simulink model "FSC_SCHEME"  (R2024b)
settings: Solver=FixedStepAuto  StartTime=0.0  StopTime=inf  FixedStep=0.001  RelTol=1e-3  EnableMultiTasking=on
libraries: px4Sensorslib x2, px4Peripheralslib x1
settings Model: SimulationMode=external  ExtModeTrigDuration=10  Creator=ArriGE66  LastModifiedBy=xippa
settings SolverCC: PositivePriorityOrder=on
settings OptimizationCC: EnhancedBackFolding=on  PassReuseOutputArgsAs=Individual arguments  ZeroExternalMemoryAtStartup=off  ZeroInternalMemoryAtStartup=off  MaxStackSize=64  OptimizeBlockOrder=speed  DifferentSizesBufferReuse=on  OptimizationCustomize=off  EfficientTunableParamExpr=on
settings DebuggingCC: ParameterTunabilityLossMsg=error
settings HardwareCC: ProdBitPerPointer=32  ProdBitPerSizeT=32  ProdBitPerPtrDiffT=32  ProdLargestAtomicInteger=Long  ProdLargestAtomicFloat=Double  ProdWordSize=32  ProdLongLongMode=on  ProdHWDeviceType=ARM Compatible->ARM Cortex
settings SFSimCC: MATLABDynamicMemAlloc=off  SimTargetLang=C++
settings RTWCC: Description=Embedded Coder  SystemTargetFile=ert.tlc  HardwareBoard=PX4 Cube Orange  TemplateMakefile=ert_default_tmf  Toolchain=GNU Tools for PX4 Autopilots  TargetLang=C++  GPUComputeCapability=3.5
settings CodeAppCC: ForceParamTrailComments=on  IgnoreCustomStorageClasses=off  OperatorAnnotations=on  SimulinkDataObjDesc=on  SFDataObjDesc=on  InsertBlockDesc=on
settings ERTTargetCC: SupportVariableSizeSignals=on  ExtMode=on  ExtModeTransport=3  ExtModeStaticAlloc=on  ExtModeStaticAllocSize=1024  ExtModeMexFile=ext_xcp  ExtModeMexArgs=1 COM10 3000000  ExtModeIntrfLevel=Level2 - Open  InlinedParameterPlacement=Hierarchical  DynamicArrayContainerType=coder::array

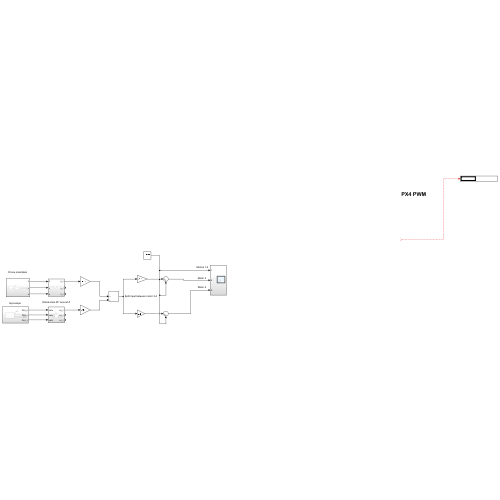
[thumbnail: Simulink's stored preview of the top-level diagram]
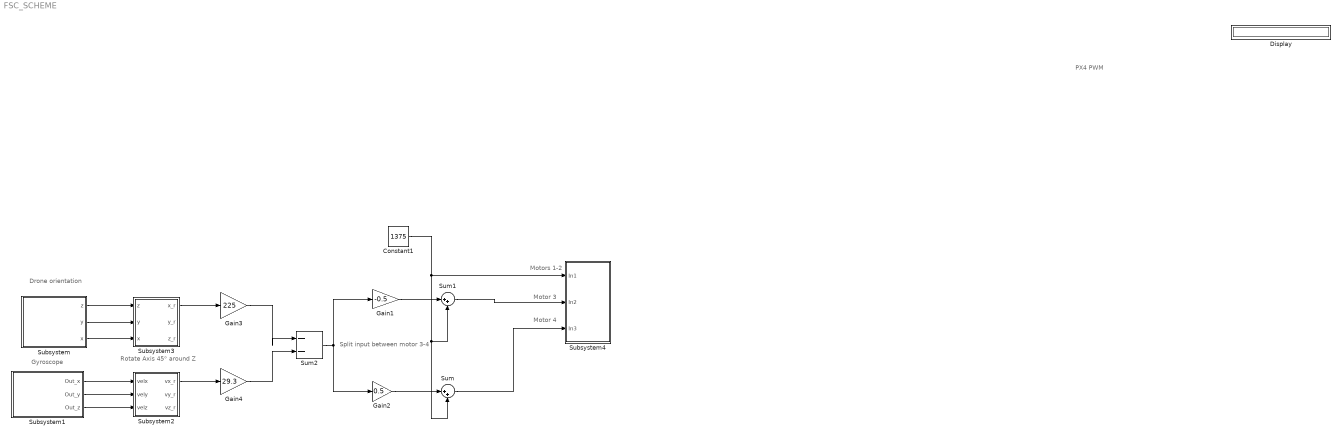
== system FSC_SCHEME ==
  note: Motor 4
  note: Motor 3
  note: Motors 1-2
  note: Split input between motor 3-4
  note: Rotate Axis 45° around Z
  note: Gyroscope
  note: Drone orientation
  note: PX4 PWM
  Constant1 : Constant  Value=1375  SampleTime=0.001
  Display : Display
      settings: Format=binary (Stored Integer)
  Gain1 : Gain  Gain=-0.5
  Gain2 : Gain  Gain=0.5
  Gain3 : Gain  Gain=225
  Gain4 : Gain  Gain=29.3
  Subsystem : Subsystem
  Subsystem1 : Subsystem
  Subsystem2 : Subsystem
  Subsystem3 : Subsystem
  Subsystem4 : Subsystem
  Sum : Sum  Inputs=|++
  Sum1 : Sum  Inputs=|++
  Sum2 : Sum  Inputs=|--
  wires:
  Gain1/1 -> Sum1/1
  Gain2/1 -> Sum/1
  ? -> Display/1
  Constant1/1 -> Sum1/2, Sum/2, Subsystem4/1(In1)
  Sum2/1 -> Gain2/1, Gain1/1
  Gain3/1 -> Sum2/1
  Gain4/1 -> Sum2/2
  Subsystem2/1(vx_r) -> Gain4/1
  Subsystem1/1(Out_x) -> Subsystem2/1(velx)
  Subsystem1/2(Out_y) -> Subsystem2/2(vely)
  Subsystem1/3(Out_z) -> Subsystem2/3(velz)
  Subsystem3/1(x_r) -> Gain3/1
  Subsystem/1(z) -> Subsystem3/1(z)
  Subsystem/2(y) -> Subsystem3/2(y)
  Subsystem/3(x) -> Subsystem3/3(x)
  Sum1/1 -> Subsystem4/2(In2)
  Sum/1 -> Subsystem4/3(In3)

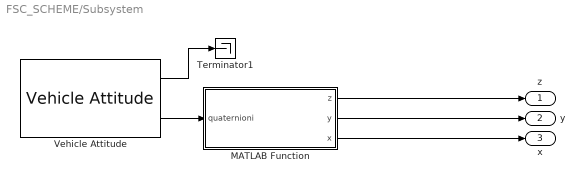
== system FSC_SCHEME/Subsystem ==
  MATLAB Function : MATLAB Function  TreatAsAtomicUnit=on
  Terminator1 : Terminator
  Vehicle Attitude : px4Sensorslib/Vehicle Attitude  rollRate=off  pitchRate=off  yawRate=off  quaternion=on  uorbTimeStamp=off  BlockingMode=off  BlockTimeout=0.001  sampleTime=1/50
  z : Outport
  y : Outport  Port=2
  x : Outport  Port=3
  wires:
  MATLAB Function/2(y) -> y/1
  Vehicle Attitude/2 -> MATLAB Function/1(quaternioni)
  MATLAB Function/3(x) -> x/1
  Vehicle Attitude/1 -> Terminator1/1
  MATLAB Function/1(z) -> z/1

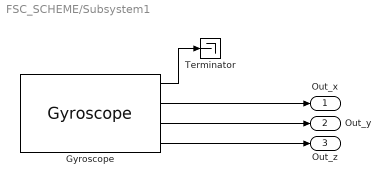
== system FSC_SCHEME/Subsystem1 ==
  Gyroscope : px4Sensorslib/Gyroscope  uorbTimeStamp=off  BlockingMode=off  BlockTimeout=1e-3  sampleTime=1/50
  Terminator : Terminator
  Out_x : Outport
  Out_y : Outport  Port=2
  Out_z : Outport  Port=3
  wires:
  Gyroscope/1 -> Terminator/1
  Gyroscope/4 -> Out_z/1
  Gyroscope/3 -> Out_y/1
  Gyroscope/2 -> Out_x/1

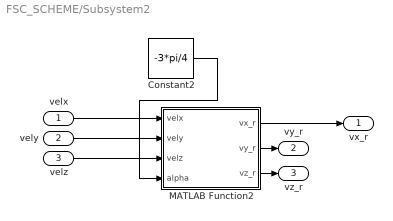
== system FSC_SCHEME/Subsystem2 ==
  velx : Inport
  vely : Inport  Port=2
  velz : Inport  Port=3
  Constant2 : Constant  Value=-3*pi/4
  MATLAB Function2 : MATLAB Function  TreatAsAtomicUnit=on
  vx_r : Outport
  vy_r : Outport  Port=2
  vz_r : Outport  Port=3
  wires:
  velz/1 -> MATLAB Function2/3(velz)
  velx/1 -> MATLAB Function2/1(velx)
  Constant2/1 -> MATLAB Function2/4(alpha)
  vely/1 -> MATLAB Function2/2(vely)
  MATLAB Function2/1(vx_r) -> vx_r/1
  MATLAB Function2/2(vy_r) -> vy_r/1
  MATLAB Function2/3(vz_r) -> vz_r/1

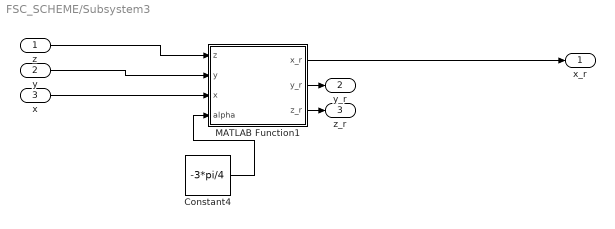
== system FSC_SCHEME/Subsystem3 ==
  z : Inport
  y : Inport  Port=2
  x : Inport  Port=3
  Constant4 : Constant  Value=-3*pi/4
  MATLAB Function1 : MATLAB Function  TreatAsAtomicUnit=on
  x_r : Outport
  y_r : Outport  Port=2
  z_r : Outport  Port=3
  wires:
  Constant4/1 -> MATLAB Function1/4(alpha)
  MATLAB Function1/3(z_r) -> z_r/1
  MATLAB Function1/2(y_r) -> y_r/1
  z/1 -> MATLAB Function1/1(z)
  MATLAB Function1/1(x_r) -> x_r/1
  y/1 -> MATLAB Function1/2(y)
  x/1 -> MATLAB Function1/3(x)

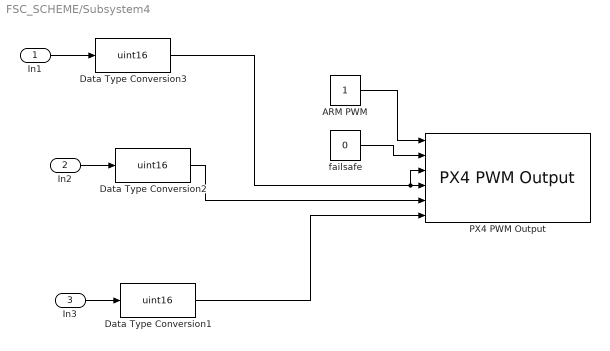
== system FSC_SCHEME/Subsystem4 ==
  In1 : Inport
  In2 : Inport  Port=2
  In3 : Inport  Port=3
  ARM PWM : Constant  OutDataTypeStr=boolean  SampleTime=0.001
  Data Type Conversion1 : DataTypeConversion  OutDataTypeStr=uint16  SaturateOnIntegerOverflow=off  RndMeth=Floor
  Data Type Conversion2 : DataTypeConversion  OutDataTypeStr=uint16  SaturateOnIntegerOverflow=off  RndMeth=Floor
  Data Type Conversion3 : DataTypeConversion  OutDataTypeStr=uint16  SaturateOnIntegerOverflow=off  RndMeth=Floor
  PX4 PWM Output : px4Peripheralslib/PX4 PWM Output  pwmDevice=Main  pwmChannel1_=on  pwmChannel2_=on  pwmChannel3_=on  pwmChannel4_=on  pwmChannel5_=off  pwmChannel6_=off  pwmChannel7_=off  pwmChannel8_=off
  failsafe : Constant  Value=0  OutDataTypeStr=boolean  SampleTime=0.001
  wires:
  failsafe/1 -> PX4 PWM Output/2
  Data Type Conversion3/1 -> PX4 PWM Output/3, PX4 PWM Output/4
  ARM PWM/1 -> PX4 PWM Output/1
  Data Type Conversion2/1 -> PX4 PWM Output/5
  Data Type Conversion1/1 -> PX4 PWM Output/6
  In2/1 -> Data Type Conversion2/1
  In3/1 -> Data Type Conversion1/1
  In1/1 -> Data Type Conversion3/1

== matlab function FSC_SCHEME/Subsystem3/MATLAB Function1 ==
  data: z input; y input; x input; x_r output; alpha input; y_r output; z_r output
function [x_r,y_r,z_r] = ruoto(z,y,x,alpha)
Global_POV = [x y z];
R_z = [cos(alpha), -sin(alpha), 0;
       sin(alpha), cos(alpha), 0;
       0, 0, 1];
LOCALPOV = Global_POV * R_z;
x_r = LOCALPOV(1);
y_r = LOCALPOV(2);
z_r = LOCALPOV(3);
end

== matlab function FSC_SCHEME/Subsystem/MATLAB Function ==
  data: quaternioni input; z output; y output; x output
function [z, y, x] = fcn(quaternioni)
eulero = zeros(1,3);
eulero = quat2eul(quaternioni);
z = eulero(1);
y = eulero(2);
x = eulero(3);
end

== matlab function FSC_SCHEME/Subsystem2/MATLAB Function2 ==
  data: velx input; vely input; velz input; vx_r output; alpha input; vy_r output; vz_r output
function [vx_r,vy_r,vz_r] = ruotovel(velx,vely,velz,alpha)
Global_POV = [velx vely velz];
R_z = [cos(alpha), -sin(alpha), 0;
       sin(alpha), cos(alpha), 0;
       0, 0, 1];
LOCALPOV = Global_POV * R_z;
vx_r = LOCALPOV(1);
vy_r = LOCALPOV(2);
vz_r = LOCALPOV(3);
end
